simulink model "FullFMS - 2025-11-05 - V0.1"  (R2025b)
settings: Solver=VariableStepAuto  StartTime=0.0  StopTime=inf  RelTol=1e-3
libraries: opcualib x2
settings Model: SimulationMode=accelerator  Creator=guilh  LastModifiedBy=gasie

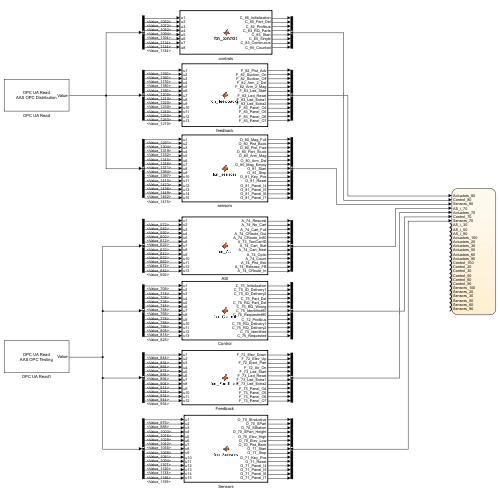
[thumbnail: Simulink's stored preview of the top-level diagram]
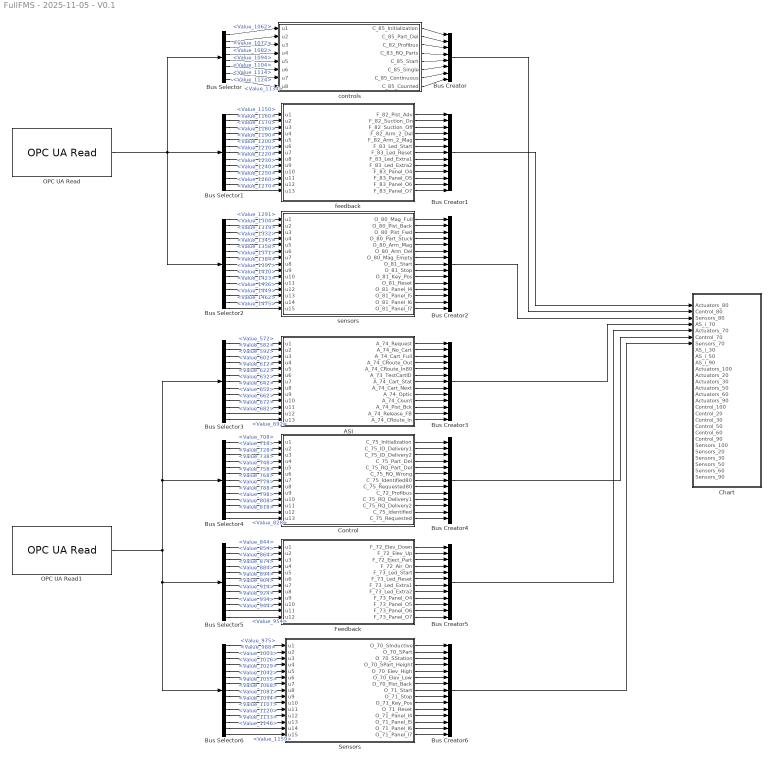
== system FullFMS - 2025-11-05 - V0.1 ==
  ASI : MATLAB Function  TreatAsAtomicUnit=on
  Bus Creator : BusCreator  Inputs=8
  Bus Creator1 : BusCreator  Inputs=13
  Bus Creator2 : BusCreator  Inputs=15
  Bus Creator3 : BusCreator  Inputs=13
  Bus Creator4 : BusCreator  Inputs=13
  Bus Creator5 : BusCreator  Inputs=12
  Bus Creator6 : BusCreator  Inputs=15
  Bus Selector : BusSelector  OutputSignals=Value_1062,Value_1072,Value_1082,Value_1094,Value_1104,Value_1114,Value_1124,Value_1134
  Bus Selector1 : BusSelector  OutputSignals=Value_1150,Value_1160,Value_1170,Value_1180,Value_1190,Value_1200,Value_1210,Value_1220,Value_1230,Value_1240,Value_1250,Value_1260,Value_1270
  Bus Selector2 : BusSelector  OutputSignals=Value_1291,Value_1304,Value_1319,Value_1332,Value_1345,Value_1358,Value_1371,Value_1384,Value_1397,Value_1410,Value_1423,Value_1436,Value_1449,Value_1462,Value_1475
  Bus Selector3 : BusSelector  OutputSignals=Value_572,Value_582,Value_592,Value_602,Value_612,Value_622,Value_632,Value_642,Value_652,Value_662,Value_672,Value_682,Value_692
  Bus Selector4 : BusSelector  OutputSignals=Value_708,Value_718,Value_728,Value_738,Value_748,Value_758,Value_768,Value_778,Value_788,Value_798,Value_808,Value_818,Value_828
  Bus Selector5 : BusSelector  OutputSignals=Value_844,Value_854,Value_864,Value_874,Value_884,Value_894,Value_904,Value_914,Value_924,Value_934,Value_944,Value_954
  Bus Selector6 : BusSelector  OutputSignals=Value_975,Value_988,Value_1003,Value_1016,Value_1029,Value_1042,Value_1055,Value_1068,Value_1081,Value_1094,Value_1107,Value_1120,Value_1133,Value_1146,Value_1159
  Chart : Stateflow chart  TreatAsAtomicUnit=on
      settings: PortSchema="{\"entries\":[{\"content\":{\"sides\":[{\"content\":{\"connectorIds\":[\"In2\",\"In1\",\"In3\",\"In4\",\"In6\",\"In5\",\"In7\",\"In8\",\"In9\",\"In10\",\"In11\",\"In12\",\"In13\",\"In14\",\"In15\",\"In16\",\"In17\",\"In18\",\"In19\",\"In20\",\"In21\",\"In22\",\"In23\",\"In24\",\"In25\",\"In26\",\"In27\",\"In28\"]},\"type\":\"ConnectorPlacement.EquallySpacedRectSide\",\"uuid\":\"e54bf7d4-7c7d-41d9-a8b8-f479ac319a99\"},{\"content\":{\"side\":\"RIGHT\"},\"type\":\"ConnectorPlacement.EquallySpacedRectSide\",\"uuid\":\"d3c20706-71bd-4e26-b40f-0ee7e71b06ee\"},{\"content\":{\"side\":\"TOP\"},\"type\":\"ConnectorPlacement.EquallySpacedRectSide\",\"uuid\":\"ecfb6920-e95b-4ed8-99f9-df5ce878328e\"}]},\"type\":\"ConnectorPlacement.EquallySpacedConnector\",\"uuid\":\"2e714192-4eea-4e1a-8945-7c827feed48f\"}],\"packageUris\":[\"http://schema.mathworks.com/mf0/Connector/R2020b\"],\"version\":\"1.0\"}"
  Control : MATLAB Function  TreatAsAtomicUnit=on
  Feedback : MATLAB Function  TreatAsAtomicUnit=on
  OPC UA Read : opcualib/OPC UA Read  SelectedServer=AAS OPC Distribution  ServerList=AAS OPC Distribution  NodeList={ '1', 'Value', '6', '1062', '1'; '2', 'Value', '6', '1072', '1'; '3', 'Value', '6', '1082', '1'; '4', 'Value', '6', '1094', '1'; '5', 'Value', '6', '1104', '1'; '6', 'Value', '6', '1114', '1'; '7', 'Value', '6', '1124', '1'; '8', 'Value', '6', '1134', '1'; '9', 'Value', '6', '1150', '1'; '10', 'Value', '6', '1160', '1'; '11', 'Value', '6', '1170', '1'; '12', 'Value', '6', '1180', '1'; '13', 'Value', '6', '1190', '1'; '14', 'Value', '6', '1200', '1'; '15', 'Value', '6', '1210', '1'; '16', 'Value', '6', '1220', '1'; '17', 'Value', '6', '1230', '1'; '18', 'Value', '6', '1240', '1'; '19', 'Value', '6', '1250', '1'; '20', 'Value', '6', '1260', '1'; '21', 'Value', '6', '1270', '1'; '22', 'Value', '6', '1291', '1'; '23', 'Value', '6', '1304', '1'; '24', 'Value', '6', '1319', '1'; '25', 'Value', '6', '1332', '1'; '26', 'Value', '6', '1345', '1'; '27', 'Value', '6', '1358', '1'; '28', 'Value', '6', '1371', '1'; '29', 'Value', '6', '1384', '1'; '30', 'Value', '6', '1397', '1'; '31', 'Value', '6', '1410', '1'; '32', 'Value', '6', '1423', '1'; '33', 'Value', '6', '1436', '1'; '34', 'Value', '6', '1449', '1'; '35', 'Value', '6', '1462', '1'; '36', 'Value', '6', '1475', '1' }  ShowQualityPort=off  ShowTimestampPort=off  ShowTimestampPortAs=Seconds since start  SampleTime=-1
  OPC UA Read1 : opcualib/OPC UA Read  SelectedServer=AAS OPC Testing  ServerList=AAS OPC Testing  NodeList={ '1', 'Value', '6', '572', '1'; '2', 'Value', '6', '582', '1'; '3', 'Value', '6', '592', '1'; '4', 'Value', '6', '602', '1'; '5', 'Value', '6', '612', '1'; '6', 'Value', '6', '622', '1'; '7', 'Value', '6', '632', '1'; '8', 'Value', '6', '642', '1'; '9', 'Value', '6', '652', '1'; '10', 'Value', '6', '662', '1'; '11', 'Value', '6', '672', '1'; '12', 'Value', '6', '682', '1'; '13', 'Value', '6', '692', '1'; '14', 'Value', '6', '708', '1'; '15', 'Value', '6', '718', '1'; '16', 'Value', '6', '728', '1'; '17', 'Value', '6', '738', '1'; '18', 'Value', '6', '748', '1'; '19', 'Value', '6', '758', '1'; '20', 'Value', '6', '768', '1'; '21', 'Value', '6', '778', '1'; '22', 'Value', '6', '788', '1'; '23', 'Value', '6', '798', '1'; '24', 'Value', '6', '808', '1'; '25', 'Value', '6', '818', '1'; '26', 'Value', '6', '828', '1'; '27', 'Value', '6', '844', '1'; '28', 'Value', '6', '854', '1'; '29', 'Value', '6', '864', '1'; '30', 'Value', '6', '874', '1'; '31', 'Value', '6', '884', '1'; '32', 'Value', '6', '894', '1'; '33', 'Value', '6', '904', '1'; '34', 'Value', '6', '914', '1'; '35', 'Value', '6', '924', '1'; '36', 'Value', '6', '934', '1'; '37', 'Value', '6', '944', '1'; '38', 'Value', '6', '954', '1'; '39', 'Value', '6', '975', '1'; '40', 'Value', '6', '988', '1'; '41', 'Value', '6', '1003', '1'; '42', 'Value', '6', '1016', '1'; '43', 'Value', '6', '1029', '1'; '44', 'Value', '6', '1042', '1'; '45', 'Value', '6', '1055', '1'; '46', 'Value', '6', '1068', '1'; '47', 'Value', '6', '1081', '1'; '48', 'Value', '6', '1094', '1'; '49', 'Value', '6', '1107', '1'; '50', 'Value', '6', '1120', '1'; '51', 'Value', '6', '1133', '1'; '52', 'Value', '6', '1146', '1'; '53', 'Value', '6', '1159', '1' }  ShowQualityPort=off  ShowTimestampPort=off  ShowTimestampPortAs=Seconds since start  SampleTime=-1
  Sensors : MATLAB Function  TreatAsAtomicUnit=on
  controls : MATLAB Function  TreatAsAtomicUnit=on
  feedback : MATLAB Function  TreatAsAtomicUnit=on
  sensors : MATLAB Function  TreatAsAtomicUnit=on
  wires:
  OPC UA Read/1 -> Bus Selector2/1, Bus Selector/1, Bus Selector1/1
  Bus Selector/1 -> controls/1(u1)  "<Value_1062>"
  Bus Selector/2 -> controls/2(u2)  "<Value_1072>"
  Bus Selector/3 -> controls/3(u3)  "<Value_1082>"
  Bus Selector/4 -> controls/4(u4)  "<Value_1094>"
  Bus Selector/5 -> controls/5(u5)  "<Value_1104>"
  Bus Selector/6 -> controls/6(u6)  "<Value_1114>"
  Bus Selector/7 -> controls/7(u7)  "<Value_1124>"
  Bus Selector/8 -> controls/8(u8)  "<Value_1134>"
  Bus Selector1/11 -> feedback/11(u11)  "<Value_1250>"
  Bus Selector1/12 -> feedback/12(u12)  "<Value_1260>"
  Bus Selector1/13 -> feedback/13(u13)  "<Value_1270>"
  Bus Selector1/1 -> feedback/1(u1)  "<Value_1150>"
  Bus Selector1/2 -> feedback/2(u2)  "<Value_1160>"
  Bus Selector1/3 -> feedback/3(u3)  "<Value_1170>"
  Bus Selector1/4 -> feedback/4(u4)  "<Value_1180>"
  Bus Selector1/5 -> feedback/5(u5)  "<Value_1190>"
  Bus Selector1/6 -> feedback/6(u6)  "<Value_1200>"
  Bus Selector1/7 -> feedback/7(u7)  "<Value_1210>"
  Bus Selector1/8 -> feedback/8(u8)  "<Value_1220>"
  Bus Selector1/9 -> feedback/9(u9)  "<Value_1230>"
  Bus Selector1/10 -> feedback/10(u10)  "<Value_1240>"
  Bus Selector2/1 -> sensors/1(u1)  "<Value_1291>"
  Bus Selector2/2 -> sensors/2(u2)  "<Value_1304>"
  Bus Selector2/3 -> sensors/3(u3)  "<Value_1319>"
  Bus Selector2/4 -> sensors/4(u4)  "<Value_1332>"
  Bus Selector2/5 -> sensors/5(u5)  "<Value_1345>"
  Bus Selector2/6 -> sensors/6(u6)  "<Value_1358>"
  Bus Selector2/7 -> sensors/7(u7)  "<Value_1371>"
  Bus Selector2/8 -> sensors/8(u8)  "<Value_1384>"
  Bus Selector2/9 -> sensors/9(u9)  "<Value_1397>"
  Bus Selector2/10 -> sensors/10(u10)  "<Value_1410>"
  Bus Selector2/11 -> sensors/11(u11)  "<Value_1423>"
  Bus Selector2/12 -> sensors/12(u12)  "<Value_1436>"
  Bus Selector2/13 -> sensors/13(u13)  "<Value_1449>"
  Bus Selector2/14 -> sensors/14(u14)  "<Value_1462>"
  Bus Selector2/15 -> sensors/15(u15)  "<Value_1475>"
  OPC UA Read1/1 -> Bus Selector6/1, Bus Selector5/1, Bus Selector3/1, Bus Selector4/1
  Bus Selector3/1 -> ASI/1(u1)  "<Value_572>"
  Bus Selector3/2 -> ASI/2(u2)  "<Value_582>"
  Bus Selector3/3 -> ASI/3(u3)  "<Value_592>"
  Bus Selector3/4 -> ASI/4(u4)  "<Value_602>"
  Bus Selector3/5 -> ASI/5(u5)  "<Value_612>"
  Bus Selector3/6 -> ASI/6(u6)  "<Value_622>"
  Bus Selector3/7 -> ASI/7(u7)  "<Value_632>"
  Bus Selector3/8 -> ASI/8(u8)  "<Value_642>"
  Bus Selector3/9 -> ASI/9(u9)  "<Value_652>"
  Bus Selector3/10 -> ASI/10(u10)  "<Value_662>"
  Bus Selector3/11 -> ASI/11(u11)  "<Value_672>"
  Bus Selector3/12 -> ASI/12(u12)  "<Value_682>"
  Bus Selector3/13 -> ASI/13(u13)  "<Value_692>"
  Bus Selector4/1 -> Control/1(u1)  "<Value_708>"
  Bus Selector4/2 -> Control/2(u2)  "<Value_718>"
  Bus Selector4/3 -> Control/3(u3)  "<Value_728>"
  Bus Selector4/4 -> Control/4(u4)  "<Value_738>"
  Bus Selector4/5 -> Control/5(u5)  "<Value_748>"
  Bus Selector4/6 -> Control/6(u6)  "<Value_758>"
  Bus Selector4/7 -> Control/7(u7)  "<Value_768>"
  Bus Selector4/8 -> Control/8(u8)  "<Value_778>"
  Bus Selector4/9 -> Control/9(u9)  "<Value_788>"
  Bus Selector4/10 -> Control/10(u10)  "<Value_798>"
  Bus Selector4/11 -> Control/11(u11)  "<Value_808>"
  Bus Selector4/12 -> Control/12(u12)  "<Value_818>"
  Bus Selector4/13 -> Control/13(u13)  "<Value_828>"
  Bus Selector5/1 -> Feedback/1(u1)  "<Value_844>"
  Bus Selector5/2 -> Feedback/2(u2)  "<Value_854>"
  Bus Selector5/3 -> Feedback/3(u3)  "<Value_864>"
  Bus Selector5/4 -> Feedback/4(u4)  "<Value_874>"
  Bus Selector5/5 -> Feedback/5(u5)  "<Value_884>"
  Bus Selector5/6 -> Feedback/6(u6)  "<Value_894>"
  Bus Selector5/7 -> Feedback/7(u7)  "<Value_904>"
  Bus Selector5/8 -> Feedback/8(u8)  "<Value_914>"
  Bus Selector5/9 -> Feedback/9(u9)  "<Value_924>"
  Bus Selector5/10 -> Feedback/10(u10)  "<Value_934>"
  Bus Selector5/11 -> Feedback/11(u11)  "<Value_944>"
  Bus Selector5/12 -> Feedback/12(u12)  "<Value_954>"
  Bus Selector6/1 -> Sensors/1(u1)  "<Value_975>"
  Bus Selector6/2 -> Sensors/2(u2)  "<Value_988>"
  Bus Selector6/3 -> Sensors/3(u3)  "<Value_1003>"
  Bus Selector6/4 -> Sensors/4(u4)  "<Value_1016>"
  Bus Selector6/5 -> Sensors/5(u5)  "<Value_1029>"
  Bus Selector6/6 -> Sensors/6(u6)  "<Value_1042>"
  Bus Selector6/7 -> Sensors/7(u7)  "<Value_1055>"
  Bus Selector6/8 -> Sensors/8(u8)  "<Value_1068>"
  Bus Selector6/9 -> Sensors/9(u9)  "<Value_1081>"
  Bus Selector6/10 -> Sensors/10(u10)  "<Value_1094>"
  Bus Selector6/11 -> Sensors/11(u11)  "<Value_1107>"
  Bus Selector6/12 -> Sensors/12(u12)  "<Value_1120>"
  Bus Selector6/13 -> Sensors/13(u13)  "<Value_1133>"
  Bus Selector6/14 -> Sensors/14(u14)  "<Value_1146>"
  Bus Selector6/15 -> Sensors/15(u15)  "<Value_1159>"
  controls/1(C_85_Initialization) -> Bus Creator/1
  controls/2(C_85_Part_Del) -> Bus Creator/2
  controls/3(C_82_Profibus) -> Bus Creator/3
  controls/4(C_83_RQ_Parts) -> Bus Creator/4
  controls/5(C_85_Start) -> Bus Creator/5
  controls/6(C_85_Single) -> Bus Creator/6
  controls/7(C_85_Continuous) -> Bus Creator/7
  controls/8(C_85_Counted) -> Bus Creator/8
  feedback/1(F_82_Pist_Adv) -> Bus Creator1/1
  feedback/2(F_82_Suction_On) -> Bus Creator1/2
  feedback/3(F_82_Suction_Off) -> Bus Creator1/3
  feedback/4(F_82_Arm_2_Del) -> Bus Creator1/4
  feedback/5(F_82_Arm_2_Mag) -> Bus Creator1/5
  feedback/6(F_83_Led_Start) -> Bus Creator1/6
  feedback/7(F_83_Led_Reset) -> Bus Creator1/7
  feedback/8(F_83_Led_Extra1) -> Bus Creator1/8
  feedback/9(F_83_Led_Extra2) -> Bus Creator1/9
  feedback/10(F_83_Panel_O4) -> Bus Creator1/10
  feedback/11(F_83_Panel_O5) -> Bus Creator1/11
  feedback/12(F_83_Panel_O6) -> Bus Creator1/12
  feedback/13(F_83_Panel_O7) -> Bus Creator1/13
  sensors/1(O_80_Mag_Full) -> Bus Creator2/1
  sensors/2(O_80_Pist_Back) -> Bus Creator2/2
  sensors/3(O_80_Pist_Fwd) -> Bus Creator2/3
  sensors/4(O_80_Part_Stuck) -> Bus Creator2/4
  sensors/5(O_80_Arm_Mag) -> Bus Creator2/5
  sensors/6(O_80_Arm_Del) -> Bus Creator2/6
  sensors/7(O_80_Mag_Empty) -> Bus Creator2/7
  sensors/8(O_81_Start) -> Bus Creator2/8
  sensors/9(O_81_Stop) -> Bus Creator2/9
  sensors/10(O_81_Key_Pos) -> Bus Creator2/10
  sensors/11(O_81_Reset) -> Bus Creator2/11
  sensors/12(O_81_Panel_I4) -> Bus Creator2/12
  sensors/13(O_81_Panel_I5) -> Bus Creator2/13
  sensors/14(O_81_Panel_I6) -> Bus Creator2/14
  sensors/15(O_81_Panel_I7) -> Bus Creator2/15
  ASI/1(A_74_Request) -> Bus Creator3/1
  ASI/2(A_74_No_Cart) -> Bus Creator3/2
  ASI/3(A_74_Cart_Full) -> Bus Creator3/3
  ASI/4(A_74_CRoute_Out) -> Bus Creator3/4
  ASI/5(A_74_CRoute_In80) -> Bus Creator3/5
  ASI/6(A_73_TestCartID) -> Bus Creator3/6
  ASI/7(A_74_Cart_Stat) -> Bus Creator3/7
  ASI/8(A_74_Cart_Next) -> Bus Creator3/8
  ASI/9(A_74_Optic) -> Bus Creator3/9
  ASI/10(A_74_Count) -> Bus Creator3/10
  ASI/11(A_74_Pist_Bck) -> Bus Creator3/11
  ASI/12(A_74_Release_FB) -> Bus Creator3/12
  ASI/13(A_74_CRoute_In) -> Bus Creator3/13
  Control/1(C_75_Initialization) -> Bus Creator4/1
  Control/2(C_75_ID_Delivery1) -> Bus Creator4/2
  Control/3(C_75_ID_Delivery2) -> Bus Creator4/3
  Control/4(C_75_Part_Del) -> Bus Creator4/4
  Control/5(C_75_RQ_Part_Del) -> Bus Creator4/5
  Control/6(C_75_RQ_Wrong) -> Bus Creator4/6
  Control/7(C_75_Identified80) -> Bus Creator4/7
  Control/8(C_75_Requested80) -> Bus Creator4/8
  Control/9(C_72_Profibus) -> Bus Creator4/9
  Control/10(C_75_RQ_Delivery1) -> Bus Creator4/10
  Control/11(C_75_RQ_Delivery2) -> Bus Creator4/11
  Control/12(C_75_Identified) -> Bus Creator4/12
  Control/13(C_75_Requested) -> Bus Creator4/13
  Feedback/1(F_72_Elev_Down) -> Bus Creator5/1
  Feedback/2(F_72_Elev_Up) -> Bus Creator5/2
  Feedback/3(F_72_Eject_Part) -> Bus Creator5/3
  Feedback/4(F_72_Air_On) -> Bus Creator5/4
  Feedback/5(F_73_Led_Start) -> Bus Creator5/5
  Feedback/6(F_73_Led_Reset) -> Bus Creator5/6
  Feedback/7(F_73_Led_Extra1) -> Bus Creator5/7
  Feedback/8(F_73_Led_Extra2) -> Bus Creator5/8
  Feedback/9(F_73_Panel_O4) -> Bus Creator5/9
  Feedback/10(F_73_Panel_O5) -> Bus Creator5/10
  Feedback/11(F_73_Panel_O6) -> Bus Creator5/11
  Feedback/12(F_73_Panel_O7) -> Bus Creator5/12
  Sensors/1(O_70_SInductive) -> Bus Creator6/1
  Sensors/2(O_70_SPart) -> Bus Creator6/2
  Sensors/3(O_70_SStation) -> Bus Creator6/3
  Sensors/4(O_70_SPart_Height) -> Bus Creator6/4
  Sensors/5(O_70_Elev_High) -> Bus Creator6/5
  Sensors/6(O_70_Elev_Low) -> Bus Creator6/6
  Sensors/7(O_70_Pist_Back) -> Bus Creator6/7
  Sensors/8(O_71_Start) -> Bus Creator6/8
  Sensors/9(O_71_Stop) -> Bus Creator6/9
  Sensors/10(O_71_Key_Pos) -> Bus Creator6/10
  Sensors/11(O_71_Reset) -> Bus Creator6/11
  Sensors/12(O_71_Panel_I4) -> Bus Creator6/12
  Sensors/13(O_71_Panel_I5) -> Bus Creator6/13
  Sensors/14(O_71_Panel_I6) -> Bus Creator6/14
  Sensors/15(O_71_Panel_I7) -> Bus Creator6/15
  Bus Creator/1 -> Chart/1(Control_80)
  Bus Creator1/1 -> Chart/2(Actuators_80)
  Bus Creator2/1 -> Chart/3(Sensors_80)
  Bus Creator6/1 -> Chart/7(Sensors_70)
  Bus Creator5/1 -> Chart/6(Actuators_70)
  Bus Creator4/1 -> Chart/5(Control_70)
  Bus Creator3/1 -> Chart/4(AS_i_70)

== matlab function FullFMS - 2025-11-05 - V0.1/feedback ==
  data: u1 input; F_82_Pist_Adv output; u2 input; u3 input; u4 input; u5 input; u6 input; u7 input; u8 input; u9 input; u10 input; u11 input; u12 input; u13 input; F_82_Suction_On output; F_82_Suction_Off output; F_82_Arm_2_Del output; F_82_Arm_2_Mag output; F_83_Led_Start output; F_83_Led_Reset output; F_83_Led_Extra1 output; F_83_Led_Extra2 output; F_83_Panel_O4 output; F_83_Panel_O5 output; F_83_Panel_O6 output; F_83_Panel_O7 output
function [F_82_Pist_Adv,F_82_Suction_On,F_82_Suction_Off,F_82_Arm_2_Del, ...
    F_82_Arm_2_Mag,F_83_Led_Start,F_83_Led_Reset,F_83_Led_Extra1,...
    F_83_Led_Extra2,F_83_Panel_O4,F_83_Panel_O5,F_83_Panel_O6,...
    F_83_Panel_O7] = fcn_feedbacks(u1,u2,u3,u4,u5,u6,u7,u8,u9,...
    u10,u11,u12,u13)

F_82_Pist_Adv = u1;
F_82_Suction_On = u2;
F_82_Suction_Off = u3;
F_82_Arm_2_Del = u4;
F_82_Arm_2_Mag = u5;
F_83_Led_Start = u6;
F_83_Led_Reset = u7;
F_83_Led_Extra1 = u8;
F_83_Led_Extra2 = u9;
F_83_Panel_O4 = u10;
F_83_Panel_O5 = u11;
F_83_Panel_O6 = u12;
F_83_Panel_O7 = u13;

== matlab function FullFMS - 2025-11-05 - V0.1/controls ==
  data: C_85_Initialization output; C_85_Part_Del output; u1 input; u2 input; u3 input; u4 input; u5 input; u6 input; u7 input; C_82_Profibus output; C_83_RQ_Parts output; C_85_Start output; C_85_Single output; C_85_Continuous output; C_85_Counted output; u8 input
function [C_85_Initialization, C_85_Part_Del,...
    C_82_Profibus, C_83_RQ_Parts, ...
    C_85_Start,C_85_Single, C_85_Continuous, ...
    C_85_Counted] = fcn_controls(u1,u2,u3,u4,u5,u6,u7,u8)

C_85_Initialization = u1;
C_85_Part_Del = u2;
C_82_Profibus = u3;
C_83_RQ_Parts = u4;
C_85_Start = u5;
C_85_Single = u6; 
C_85_Continuous = u7;
C_85_Counted = u8;

== matlab function FullFMS - 2025-11-05 - V0.1/ASI ==
  data: u1 input; A_74_Request output; u2 input; u3 input; u4 input; u5 input; u6 input; u7 input; u8 input; u9 input; A_74_No_Cart output; A_74_Cart_Full output; A_74_CRoute_Out output; A_74_CRoute_In80 output; A_73_TestCartID output; A_74_Cart_Stat output; A_74_Cart_Next output; A_74_Optic output; A_74_Count output; A_74_Pist_Bck output; A_74_Release_FB output; A_74_CRoute_In output; u10 input; u11 input; u12 input; u13 input
function [A_74_Request, A_74_No_Cart, A_74_Cart_Full, A_74_CRoute_Out,...
    A_74_CRoute_In80, A_73_TestCartID, A_74_Cart_Stat, ...
          A_74_Cart_Next, A_74_Optic, A_74_Count, A_74_Pist_Bck, ...
          A_74_Release_FB,...
          A_74_CRoute_In] = fcn_Asi(u1, u2, u3, u4, u5, u6, u7, u8, u9,...
          u10, u11, u12, u13)

A_74_Request = u1;
A_74_No_Cart = u2;
A_74_Cart_Full = u3;
A_74_CRoute_Out = u4;
A_74_CRoute_In80 = u5;
A_73_TestCartID = u6;
A_74_Cart_Stat = u7;
A_74_Cart_Next = u8;
A_74_Optic = u9;
A_74_Count = u10;
A_74_Pist_Bck = u11;
A_74_Release_FB = u12;
A_74_CRoute_In = u13;

== matlab function FullFMS - 2025-11-05 - V0.1/sensors ==
  data: u1 input; u2 input; u3 input; u4 input; u5 input; u6 input; u7 input; u8 input; u9 input; u10 input; u11 input; u12 input; u13 input; u14 input; u15 input; O_80_Mag_Full output; O_80_Pist_Back output; O_80_Pist_Fwd output; O_80_Part_Stuck output; O_80_Arm_Mag output; O_80_Arm_Del output; O_80_Mag_Empty output; O_81_Start output; O_81_Stop output; O_81_Key_Pos output; O_81_Reset output; O_81_Panel_I4 output; O_81_Panel_I5 output; O_81_Panel_I6 output; O_81_Panel_I7 output
function [O_80_Mag_Full,O_80_Pist_Back,O_80_Pist_Fwd,O_80_Part_Stuck,...
    O_80_Arm_Mag,O_80_Arm_Del,O_80_Mag_Empty,O_81_Start,O_81_Stop,...
    O_81_Key_Pos,O_81_Reset,O_81_Panel_I4,O_81_Panel_I5,O_81_Panel_I6,...
    O_81_Panel_I7] = fcn_sensors(u1,u2,u3,u4,u5,u6,u7,u8,u9,...
    u10,u11,u12,u13,u14,u15)

O_80_Mag_Full = u1;
O_80_Pist_Back = u2;
O_80_Pist_Fwd = u3;
O_80_Part_Stuck = u4;
O_80_Arm_Mag = u5;
O_80_Arm_Del = u6;
O_80_Mag_Empty = u7;
O_81_Start = u8;
O_81_Stop = u9;
O_81_Key_Pos = u10;
O_81_Reset = u11;
O_81_Panel_I4 = u12;
O_81_Panel_I5 = u13;
O_81_Panel_I6 = u14;
O_81_Panel_I7 = u15;

== matlab function FullFMS - 2025-11-05 - V0.1/Control ==
  data: C_75_Initialization output; C_75_ID_Delivery1 output; C_75_ID_Delivery2 output; C_75_Part_Del output; C_75_RQ_Part_Del output; C_75_RQ_Wrong output; C_75_Identified80 output; C_75_Requested80 output; u1 input; C_72_Profibus output; u2 input; u3 input; u4 input; u5 input; u6 input; u7 input; u8 input; u9 input; u10 input; u11 input; u12 input; u13 input; C_75_RQ_Delivery1 output; C_75_RQ_Delivery2 output; C_75_Identified output; C_75_Requested output
function [C_75_Initialization, C_75_ID_Delivery1, C_75_ID_Delivery2, ...
          C_75_Part_Del, C_75_RQ_Part_Del, C_75_RQ_Wrong, C_75_Identified80, ...
          C_75_Requested80, C_72_Profibus, C_75_RQ_Delivery1, C_75_RQ_Delivery2, C_75_Identified, ...
          C_75_Requested] = fcn_Control(u1, u2, u3, u4, u5, u6, u7, u8, u9, u10, u11, u12, u13)

C_75_Initialization = u1;
C_75_ID_Delivery1 = u2;
C_75_ID_Delivery2 = u3;
C_75_Part_Del = u4;
C_75_RQ_Part_Del = u5;
C_75_RQ_Wrong = u6;
C_75_Identified80 = u7;
C_75_Requested80 = u8;
C_72_Profibus = u9;
C_75_RQ_Delivery1 = u10;
C_75_RQ_Delivery2 = u11;
C_75_Identified = u12;
C_75_Requested = u13;

== matlab function FullFMS - 2025-11-05 - V0.1/Feedback ==
  data: u1 input; F_72_Elev_Down output; u2 input; u3 input; u4 input; u5 input; u6 input; u7 input; u8 input; u9 input; u10 input; u11 input; u12 input; F_72_Elev_Up output; F_72_Eject_Part output; F_72_Air_On output; F_73_Led_Start output; F_73_Led_Reset output; F_73_Led_Extra1 output; F_73_Led_Extra2 output; F_73_Panel_O4 output; F_73_Panel_O5 output; F_73_Panel_O6 output; F_73_Panel_O7 output
function [F_72_Elev_Down, F_72_Elev_Up, F_72_Eject_Part, F_72_Air_On, ...
          F_73_Led_Start, F_73_Led_Reset, F_73_Led_Extra1, F_73_Led_Extra2, ...
          F_73_Panel_O4, F_73_Panel_O5, F_73_Panel_O6, F_73_Panel_O7] = ...
          fcn_Feedback(u1, u2, u3, u4, u5, u6, u7, u8, u9, u10, u11, u12)

F_72_Elev_Down = u1;
F_72_Elev_Up = u2;
F_72_Eject_Part = u3;
F_72_Air_On = u4;
F_73_Led_Start = u5;
F_73_Led_Reset = u6;
F_73_Led_Extra1 = u7;
F_73_Led_Extra2 = u8;
F_73_Panel_O4 = u9;
F_73_Panel_O5 = u10;
F_73_Panel_O6 = u11;
F_73_Panel_O7 = u12;

== matlab function FullFMS - 2025-11-05 - V0.1/Sensors ==
  data: u1 input; O_70_SInductive output; u2 input; u3 input; u4 input; u5 input; u6 input; u7 input; u8 input; u9 input; u10 input; u11 input; u12 input; u13 input; u14 input; u15 input; O_70_SPart output; O_70_SStation output; O_70_SPart_Height output; O_70_Elev_High output; O_70_Elev_Low output; O_70_Pist_Back output; O_71_Start output; O_71_Stop output; O_71_Key_Pos output; O_71_Reset output; O_71_Panel_I4 output; O_71_Panel_I5 output; O_71_Panel_I6 output; O_71_Panel_I7 output
function [O_70_SInductive, O_70_SPart, O_70_SStation, O_70_SPart_Height, ...
          O_70_Elev_High, O_70_Elev_Low, O_70_Pist_Back, O_71_Start, ...
          O_71_Stop, O_71_Key_Pos, O_71_Reset, O_71_Panel_I4, O_71_Panel_I5, ...
          O_71_Panel_I6, O_71_Panel_I7] = ...
          fcn_Sensors(u1, u2, u3, u4, u5, u6, u7, u8, u9, u10, ...
          u11, u12, u13, u14, u15)

O_70_SInductive = u1;
O_70_SPart = u2;
O_70_SStation = u3;
O_70_SPart_Height = u4;
O_70_Elev_High = u5;
O_70_Elev_Low = u6;
O_70_Pist_Back = u7;
O_71_Start = u8;
O_71_Stop = u9;
O_71_Key_Pos = u10;
O_71_Reset = u11;
O_71_Panel_I4 = u12;
O_71_Panel_I5 = u13;
O_71_Panel_I6 = u14;
O_71_Panel_I7 = u15;

== stateflow chart FullFMS - 2025-11-05 - V0.1/Chart ==
  state VarDeclaration_60
    entry:
    %Control_60
    C_65_Initialization = Control_60(1);
    C_65_ID_1           = Control_60(2);
    C_65_ID_2           = Control_60(3);
    C_62_Profibus       = Control_60(4);
    C_65_RBS_Output     = Control_60(5);
    C_65_RSB_Output     = Control_60(6);
    C_65_BRS_Output     = Control_60(7);
    C_65_BSR_Output     = Control_60(8);
    C_65_SRB_Output     = Control_60(9);
    C_65_SBR_Output     = Control_60(10);
    %Actuators_60
    F_62_Conveyor   = Actuators_60(1);
    F_62_P1         = Actuators_60(2);
    F_62_P2         = Actuators_60(3);
    F_62_Identify   = Actuators_60(4);
    F_63_Led_Start  = Actuators_60(5);
    F_63_Led_Reset  = Actuators_60(6);
    F_63_Led_Extra1 = Actuators_60(7);
    F_63_Led_Extra2 = Actuators_60(8);
    F_63_Panel_O4   = Actuators_60(9);
    F_63_Panel_O5   = Actuators_60(10);
    F_63_Panel_O6   = Actuators_60(11);
    F_63_Panel_O7   = Actuators_60(12);
    %Sensors_60
    O_60_SPart      = Sensors_60(1);
    O_60_Slnd       = Sensors_60(2);
    O_60_SPhoto     = Sensors_60(3);
    O_60_Part_Pass  = Sensors_60(4);
    O_60_SL1_Bck    = Sensors_60(5);
    O_60_SL1_Fwd    = Sensors_60(6);
    O_60_SL2_Bck    = Sensors_60(7);
    O_60_SL2_Fwd    = Sensors_60(8);
    O_61_Start      = Sensors_60(9);
    O_61_Stop       = Sensors_60(10);
    O_61_Key_Pos    = Sensors_60(11);
    O_61_Reset      = Sensors_60(12);
    O_61_Panel_I4   = Sensors_60(13);
    O_61_Panel_I5   = Sensors_60(14);
    O_61_Panel_I6   = Sensors_60(15);
    O_61_Panel_I7   = Sensors_60(16);
  state VarDeclaration_70
    entry:
    %AS_i_70
    A_74_Request = AS_i_70(1);
    A_74_No_Cart = AS_i_70(2);
    A_74_Cart_Full = AS_i_70(3);
    A_74_CRoute_Out = AS_i_70(4);
    A_74_CRoute_In80 = AS_i_70(5);
    A_73_TestCartID = AS_i_70(6);
    A_74_Cart_Stat = AS_i_70(7);
    A_74_Cart_Next = AS_i_70(8);
    A_74_Optic = AS_i_70(9);
    A_74_Count = AS_i_70(10);
    A_74_Pist_Bck = AS_i_70(11);
    A_74_Release_FB = AS_i_70(12);
    A_74_CRoute_In = AS_i_70(13);
    %Control_70
    C_75_Initialization = Control_70(1);
    C_75_ID_Delivery1 = Control_70(2);
    C_75_ID_Delivery2 = Control_70(3);
    C_75_Part_Del = Control_70(4);
    C_75_RQ_Part_Del = Control_70(5);
    C_75_RQ_Wrong = Control_70(6);
    C_75_Identified80 = Control_70(7);
    C_75_Requested80 = Control_70(8);
    C_72_Profibus = Control_70(9);
    C_75_RQ_Delivery1 = Control_70(10);
    C_75_RQ_Delivery2 = Control_70(11);
    C_75_Identified = Control_70(12);
    C_75_Requested = Control_70(13);
    %Actuators_70
    F_72_Elev_Down = Actuators_70(1);
    F_72_Elev_Up = Actuators_70(2);
    F_72_Eject_Part = Actuators_70(3);
    F_72_Air_On = Actuators_70(4);
    F_73_Led_Start = Actuators_70(5);
    F_73_Led_Reset = Actuators_70(6);
    F_73_Led_Extra1 = Actuators_70(7);
    F_73_Led_Extra2 = Actuators_70(8);
    F_73_Panel_O4 = Actuators_70(9);
    F_73_Panel_O5 = Actuators_70(10);
    F_73_Panel_O6 = Actuators_70(11);
    F_73_Panel_O7 = Actuators_70(12);
    %Sensors_70
    O_70_SInductive = Sensors_70(1);
    O_70_SPart = Sensors_70(2);
    O_70_SStation = Sensors_70(3);
    O_70_SPart_Height = Sensors_70(4);
    O_70_Elev_High = Sensors_70(5);
    O_70_Elev_Low = Sensors_70(6);
    O_70_Pist_Back = Sensors_70(7);
    O_71_Start = Sensors_70(8);
    O_71_Stop = Sensors_70(9);
    O_71_Key_Pos = Sensors_70(10);
    O_71_Reset = Sensors_70(11);
    O_71_Panel_I4 = Sensors_70(12);
    O_71_Panel_I5 = Sensors_70(13);
    O_71_Panel_I6 = Sensors_70(14);
    O_71_Panel_I7 = Sensors_70(15);
  state VarDeclaration_80
    entry:
    %Control_80
    C_85_Initialization = Control_80(1);
    C_85_Part_Del = Control_80(2);
    C_82_Profibus = Control_80(3);
    C_83_RQ_Parts = Control_80(4);
    C_85_Start = Control_80(5);
    C_85_Single = Control_80(6);
    C_85_Continuous = Control_80(7);
    C_85_Counted = Control_80(8);
    %Actuators_80
    F_82_Pist_Adv = Actuators_80(1);
    F_82_Suction_On = Actuators_80(2);
    F_82_Suction_Off = Actuators_80(3);
    F_82_Arm_2_Del = Actuators_80(4);
    F_82_Arm_2_Mag = Actuators_80(5);
    F_83_Led_Start = Actuators_80(6);
    F_83_Led_Reset = Actuators_80(7);
    F_83_Led_Extra1 = Actuators_80(8);
    F_83_Led_Extra2 = Actuators_80(9);
    F_83_Panel_O4 = Actuators_80(10);
    F_83_Panel_O5 = Actuators_80(11);
    F_83_Panel_O6 = Actuators_80(12);
    F_83_Panel_O7 = Actuators_80(13);
    %Sensors_80
    O_80_Mag_Full = Sensors_80(1);
    O_80_Pist_Back = Sensors_80(2);
    O_80_Pist_Fwd = Sensors_80(3);
    O_80_Part_Stuck = Sensors_80(4);
    O_80_Arm_Mag = Sensors_80(5);
    O_80_Arm_Del = Sensors_80(6);
    O_80_Mag_Empty = Sensors_80(7);
    O_81_Start = Sensors_80(8);
    O_81_Stop = Sensors_80(9);
    O_81_Key_Pos = Sensors_80(10);
    O_81_Reset = Sensors_80(11);
    O_81_Panel_I4 = Sensors_80(12);
    O_81_Panel_I5 = Sensors_80(13);
    O_81_Panel_I6 = Sensors_80(14);
    O_81_Panel_I7 = Sensors_80(15);
  state VarDeclaration_90
    entry:
    %AS_i_90
    A_94_Request    = AS_i_90(1);
    A_94_No_Cart    = AS_i_90(2);
    A_94_Cart_Full  = AS_i_90(3);
    A_94_CRoute_Out = AS_i_90(4);
    A_93_ProcCartID = AS_i_90(5);
    A_94_Cart_Stat  = AS_i_90(6);
    A_94_Cart_Next  = AS_i_90(7);
    A_94_Optic      = AS_i_90(8);
    A_94_Count      = AS_i_90(9);
    A_94_Pist_Bck   = AS_i_90(10);
    A_94_Release_FB = AS_i_90(11);
    A_94_CRoute_In  = AS_i_90(12);
    %Control_90
    C_95_Initialization = Control_90(1);
    C_95_PD_Proc        = Control_90(2);
    C_95_PD_Cart        = Control_90(3);
    C_92_Profibus       = Control_90(4);
    C_95_Start          = Control_90(5);
    C_95_Cart2Del       = Control_90(6);
    C_95_Del2Cart       = Control_90(7);
    %Actuators_90
    F_92_Claw_2_Cart = Actuators_90(1);
    F_92_Claw_2_Del  = Actuators_90(2);
    F_92_Claw_Down   = Actuators_90(3);
    F_92_Close_Claw  = Actuators_90(4);
    F_93_Led_Start   = Actuators_90(5);
    F_93_Led_Reset   = Actuators_90(6);
    F_93_Led_Extra1  = Actuators_90(7);
    F_93_Led_Extra2  = Actuators_90(8);
    F_93_Panel_O4    = Actuators_90(9);
    F_93_Panel_O5    = Actuators_90(10);
    F_93_Panel_O6    = Actuators_90(11);
    F_93_Panel_O7    = Actuators_90(12);
    %Sensors_90
    O_90_Part_Reserve = Sensors_90(1);
    O_90_Claw_Del     = Sensors_90(2);
    O_90_Claw_Cart    = Sensors_90(3);
    O_90_Claw_Reserve = Sensors_90(4);
    O_90_Claw_Low     = Sensors_90(5);
    O_90_Claw_High    = Sensors_90(6);
    O_90_Part_in_Claw = Sensors_90(7);
    O_91_Start        = Sensors_90(8);
    O_91_Stop         = Sensors_90(9);
    O_91_Key_Pos      = Sensors_90(10);
    O_91_Reset        = Sensors_90(11);
    O_91_Panel_I4     = Sensors_90(12);
    O_91_Panel_I5     = Sensors_90(13);
    O_91_Panel_I6     = Sensors_90(14);
    O_91_Panel_I7     = Sensors_90(15);
  state VarDeclaration_100
    entry:
    %Control_100
    C_105_Initialization = Control_100(1);
    C_105_Part_ready     = Control_100(2);
    C_105_Test_Ok        = Control_100(3);
    C_105_Test_Fail      = Control_100(4);
    C_102_Profibus       = Control_100(5);
    C_103_RQ_Turns       = Control_100(6);
    C_105_Start          = Control_100(7);
    C_105_Test           = Control_100(8);
    C_105_TestDrill      = Control_100(9);
    C_105_Rotation       = Control_100(10);
    %Actuators_100
    F_102_Drill_On   = Actuators_100(1);
    F_102_RT_On      = Actuators_100(2);
    F_102_Drill_Down = Actuators_100(3);
    F_102_Drill_Up   = Actuators_100(4);
    F_102_Drill_Pin  = Actuators_100(5);
    F_102_Test_Pin   = Actuators_100(6);
    F_103_Led_Start  = Actuators_100(7);
    F_103_Led_Reset  = Actuators_100(8);
    F_103_Led_Extra1 = Actuators_100(9);
    F_103_Led_Extra2 = Actuators_100(10);
    F_103_Panel_O4   = Actuators_100(11);
    F_103_Panel_O5   = Actuators_100(12);
    F_103_Panel_O6   = Actuators_100(13);
    F_103_Panel_O7   = Actuators_100(14);
    %Sensors_100
    O_100_PInit_Pos   = Sensors_100(1);
    O_100_PDrill_Pos  = Sensors_100(2);
    O_100_PTest_Pos   = Sensors_100(3);
    O_100_SDrill_High = Sensors_100(4);
    O_100_SDrill_Low  = Sensors_100(5);
    O_100_RT_Sensor   = Sensors_100(6);
    O_100_PTest_Ok    = Sensors_100(7);
    O_101_Start       = Sensors_100(8);
    O_101_Stop        = Sensors_100(9);
    O_101_Key_Pos     = Sensors_100(10);
    O_101_Reset       = Sensors_100(11);
    O_101_Panel_I4    = Sensors_100(12);
    O_101_Panel_I5    = Sensors_100(13);
    O_101_Panel_I6    = Sensors_100(14);
    O_101_Panel_I7    = Sensors_100(15);
  state VarDeclaration_50
    entry:
    %AS_i_50
    A_54_Request    = AS_i_50(1);
    A_54_No_Cart    = AS_i_50(2);
    A_54_Cart_Full  = AS_i_50(3);
    A_54_CRoute_Out = AS_i_50(4);
    A_53_SortCartID = AS_i_50(5);
    A_54_Cart_Stat  = AS_i_50(6);
    A_54_Cart_Next  = AS_i_50(7);
    A_54_Optic      = AS_i_50(8);
    A_54_Count      = AS_i_50(9);
    A_54_Pist_Bck   = AS_i_50(10);
    A_54_Release_FB = AS_i_50(11);
    A_54_CRoute_In  = AS_i_50(12);
    C_55_Start      = AS_i_50(13);
    C_55_Cart2Del   = AS_i_50(14);
    %Control_50
    C_55_Initialization = Control_50(1);
    C_55_PD_Sort        = Control_50(2);
    C_52_Profibus       = Control_50(3);
    C_55_Start          = Control_50(4);
    C_55_Cart2Del       = Control_50(5);
    %Actuators_50
    F_52_Claw_2_Del  = Actuators_50(1);
    F_52_Claw_2_Cart = Actuators_50(2);
    F_52_Claw_Down   = Actuators_50(3);
    F_52_Close_Claw  = Actuators_50(4);
    F_53_Led_Start   = Actuators_50(5);
    F_53_Led_Reset   = Actuators_50(6);
    F_53_Led_Extra1  = Actuators_50(7);
    F_53_Led_Extra2  = Actuators_50(8);
    F_53_Panel_O4    = Actuators_50(9);
    F_53_Panel_O5    = Actuators_50(10);
    F_53_Panel_O6    = Actuators_50(11);
    F_53_Panel_O7    = Actuators_50(12);
    %Sensors_50
    O_50_Part_Reserve = Sensors_50(1);
    O_50_Claw_Cart    = Sensors_50(2);
    O_50_Claw_Del     = Sensors_50(3);
    O_50_Claw_Reserve = Sensors_50(4);
    O_50_Claw_Low     = Sensors_50(5);
    O_50_Claw_High    = Sensors_50(6);
    O_50_Part_in_Claw = Sensors_50(7);
    O_51_Start        = Sensors_50(8);
    O_51_Stop         = Sensors_50(9);
    O_51_Key_Pos      = Sensors_50(10);
    O_51_Reset        = Sensors_50(11);
    O_51_Panel_I4     = Sensors_50(12);
    O_51_Panel_I5     = Sensors_50(13);
    O_51_Panel_I6     = Sensors_50(14);
    O_51_Panel_I7     = Sensors_50(15);
  state VarDeclaration_20
    entry:
    %Control_20
    C_24_CRoute_In  = Control_20(1);
    C_25_CRoute_In  = Control_20(2);
    C_26_CRoute_In  = Control_20(3);
    C_27_CRoute_In  = Control_20(4);
    C_28_CRoute_In  = Control_20(5);
    C_29_CRoute_In  = Control_20(6);
    C_24_Request    = Control_20(7);
    C_24_CartDel    = Control_20(8);
    C_24_CRoute_Out = Control_20(9);
    C_25_Request    = Control_20(10);
    C_25_CartDel    = Control_20(11);
    C_25_CRoute_Out = Control_20(12);
    C_26_Request    = Control_20(13);
    C_26_CartDel    = Control_20(14);
    C_26_CRoute_Out = Control_20(15);
    C_27_Request    = Control_20(16);
    C_27_CartDel    = Control_20(17);
    C_27_CRoute_Out = Control_20(18);
    C_28_Request    = Control_20(19);
    C_28_CartDel    = Control_20(20);
    C_28_CRoute_Out = Control_20(21);
    C_29_Request    = Control_20(22);
    C_29_CartDel    = Control_20(23);
    C_29_CRoute_Out = Control_20(24);
    %Actuators_20
    F_22_Led_On       = Actuators_20(1);
    F_22_Led_Off      = Actuators_20(2);
    F_22_Conveyor   = Actuators_20(3);
    F_24_Release_FB   = Actuators_20(4);
    F_25_Release_FB   = Actuators_20(5);
    F_26_Release_FB   = Actuators_20(6);
    F_27_Release_FB   = Actuators_20(7);
    F_28_Release_FB   = Actuators_20(8);
    F_29_Release_FB   = Actuators_20(9);
    %Sensors_20
    O_20_On            = Sensors_20(1);
    O_20_Off           = Sensors_20(2);
    O_20_Controler_On  = Sensors_20(3);
    O_24_Cart_Stat     = Sensors_20(4);
    O_24_Cart_Next     = Sensors_20(5);
    O_24_Optic         = Sensors_20(6);
    O_24_Count         = Sensors_20(7);
    O_24_Pist_Bck      = Sensors_20(8);
    O_25_Cart_Stat     = Sensors_20(9);
    O_25_Cart_Next     = Sensors_20(10);
    O_25_Optic         = Sensors_20(11);
    O_25_Count         = Sensors_20(12);
    O_25_Pist_Back     = Sensors_20(13);
    O_26_Cart_Stat     = Sensors_20(14);
    O_26_Cart_Next     = Sensors_20(15);
    O_26_Optic         = Sensors_20(16);
    O_26_Count         = Sensors_20(17);
    O_26_Pist_Back     = Sensors_20(18);
    O_27_Cart_Stat     = Sensors_20(19);
    O_27_Cart_Next     = Sensors_20(20);
    O_27_Optic         = Sensors_20(21);
    O_27_Count         = Sensors_20(22);
    O_27_Pist_Back     = Sensors_20(23);
    O_28_Cart_Stat     = Sensors_20(24);
    O_28_Cart_Next     = Sensors_20(25);
    O_28_Optic         = Sensors_20(26);
    O_28_Count         = Sensors_20(27);
    O_28_Pist_Back     = Sensors_20(28);
    O_29_Cart_Stat     = Sensors_20(29);
    O_29_Cart_Next     = Sensors_20(30);
    O_29_Optic         = Sensors_20(31);
    O_29_Count         = Sensors_20(32);
    O_29_Pist_Back     = Sensors_20(33);
  state VarDeclaration_30
    entry:
    %AS_i_30
    A_34_Request    = AS_i_30(1);
    A_34_No_Cart    = AS_i_30(2);
    A_34_Cart_Full  = AS_i_30(3);
    A_34_CRoute_Out = AS_i_30(4);
    A_32_RoboCartID = AS_i_30(5);
    A_34_Cart_Stat  = AS_i_30(6);
    A_34_Cart_Next  = AS_i_30(7);
    A_34_Optic      = AS_i_30(8);
    A_34_Count      = AS_i_30(9);
    A_34_Pist_Bck   = AS_i_30(10);
    A_34_Release_FB = AS_i_30(11);
    A_34_CRoute_In  = AS_i_30(12);
    %Control_30
    C_30_Robot1   = Control_30(1);
    C_30_Robot2   = Control_30(2);
    C_35_Part_Del = Control_30(3);
    %Actuators_30
    F_33_Led_Start  = Actuators_30(1);
    F_33_Led_Reset  = Actuators_30(2);
    F_33_Led_Extra1 = Actuators_30(3);
    F_33_Led_Extra2 = Actuators_30(4);
    F_33_Spring_Cyl = Actuators_30(5);
    F_33_Cover_Cyl  = Actuators_30(6);
    %Sensors_30
    O_31_Start        = Sensors_30(1);
    O_31_Stop         = Sensors_30(2);
    O_31_Reset        = Sensors_30(3);
    O_31_Part_in_Claw = Sensors_30(4);
    O_31_Orientation  = Sensors_30(5);
    O_32_Sp_Cyl_Bck   = Sensors_30(6);
    O_32_Sp_Cyl_Fwd   = Sensors_30(7);
    O_32_Co_Cyl_Bck   = Sensors_30(8);
    O_32_Co_Cyl_Fwd   = Sensors_30(9);
    O_32_Sp_PickUp    = Sensors_30(10);
    O_32_Co_PickUp    = Sensors_30(11);
    O_32_CoMag_Empty  = Sensors_30(12);
  state Test_Drill
    during:
    C_105_Part_ready
  state ReturnToCart
    during:
    C_95_PD_Cart
  state Start
    during:
    C_24_Request
  state CartToTesting
    during:
    C_24_CartDel
  state GetsPart
    during:
    C_85_Part_Del
  state Identifies Part
    during:
    C_75_Part_Del
    A_74_CRoute_Out
  state CartToHandling2
    during:
    C_25_CartDel
  state DeliverToProcessing
    during:
    C_95_PD_Proc
  state Test_Only
    during:
    C_105_Part_ready
  state CarrinhoParaVision
    during:
    C_26_CartDel
  state Rotation_Only
    during:
    C_105_Part_ready
  (default) -> VarDeclaration_100
  VarDeclaration_90 -> VarDeclaration_80
  VarDeclaration_50 -> VarDeclaration_30
  VarDeclaration_70 -> VarDeclaration_60
  VarDeclaration_30 -> VarDeclaration_20
  VarDeclaration_80 -> VarDeclaration_70
  VarDeclaration_60 -> VarDeclaration_50
  VarDeclaration_100 -> VarDeclaration_90
  Test_Drill -> ReturnToCart : [C_105_Part_ready == true]
  DeliverToProcessing -> Test_Drill [order 1] : [C_95_PD_Proc == true] && [C_105_TestDril == true]
  CartToTesting -> GetsPart : [C_24_CartDel == true]
  Start -> CartToTesting : [C_24_Request == true]
  GetsPart -> Identifies Part : [C_85_Part_Del == true]
  Test_Only -> ReturnToCart : [C_105_Part_ready == true]
  Rotation_Only -> ReturnToCart : [C_105_Part_ready == true]
  DeliverToProcessing -> Test_Only [order 2] : [C_95_PD_Proc == true] && [C_105_Test == true]
  ReturnToCart -> CarrinhoParaVision : [C_95_PD_Cart == true]
  CartToHandling2 -> DeliverToProcessing : [C_25_CartDel == true]
  Identifies Part -> CartToHandling2 : [C_75_Part_Del == true && A_74_CRoute_Out == true ]
  DeliverToProcessing -> Rotation_Only [order 3] : [C_95_PD_Proc == true] && [C_105_Rotation == true]
  data: Control_80 input; Actuators_80 input; Sensors_80 input; AS_i_70 input; Control_70 input; Actuators_70 input; Sensors_70 input; C_82_Profibus local; C_83_RQ_Parts local; C_85_Continuous local; C_85_Counted local; C_85_Initialization local; C_85_Part_Del local; C_85_Single local; C_85_Start local; F_82_Arm_2_Del local; F_82_Arm_2_Mag local; F_82_Pist_Adv local; F_82_Suction_Off local; F_82_Suction_On local; F_83_Led_Extra1 local; F_83_Led_Extra2 local; F_83_Led_Reset local; F_83_Led_Start local; F_83_Panel_O4 local; F_83_Panel_O5 local; F_83_Panel_O6 local; F_83_Panel_O7 local; O_80_Arm_Del local; O_80_Arm_Mag local; O_80_Mag_Empty local; O_80_Mag_Full local; O_80_Part_Stuck local; O_80_Pist_Back local; O_80_Pist_Fwd local; O_81_Key_Pos local; O_81_Panel_I4 local; O_81_Panel_I5 local; O_81_Panel_I6 local; O_81_Panel_I7 local; O_81_Reset local; O_81_Start local; O_81_Stop local; C_75_ID_Delivery1 local; C_75_ID_Delivery2 local; C_75_Identified local; C_75_Identified80 local; C_75_Initialization local; C_75_Part_Del local; C_75_RQ_Delivery1 local; C_75_RQ_Delivery2 local; C_75_RQ_Part_Del local; C_75_RQ_Wrong local; C_75_Requested local; C_75_Requested80 local; F_72_Air_On local; F_72_Eject_Part local; F_72_Elev_Down local; F_72_Elev_Up local; F_73_Led_Extra1 local; F_73_Led_Extra2 local; F_73_Led_Reset local; F_73_Led_Start local; F_73_Panel_O4 local; F_73_Panel_O5 local; F_73_Panel_O6 local; F_73_Panel_O7 local; O_70_Elev_High local; O_70_Elev_Low local; O_70_Pist_Back local; O_70_SInductive local; O_70_SPart local; O_70_SPart_Height local; O_70_SStation local; O_71_Key_Pos local; O_71_Panel_I4 local; O_71_Panel_I5 local; O_71_Panel_I6 local; O_71_Panel_I7 local; O_71_Reset local; O_71_Start local; O_71_Stop local; A_73_TestCartID local; A_74_CRoute_In local; A_74_CRoute_In80 local; A_74_CRoute_Out local; A_74_Cart_Full local; A_74_Cart_Next local; A_74_Cart_Stat local; A_74_Count local; A_74_No_Cart local; A_74_Optic local; A_74_Pist_Bck local; A_74_Release_FB local; A_74_Request local; C_72_Profibus local; AS_i_30 input; AS_i_50 input; AS_i_90 input; Actuators_100 input; Actuators_20 input; Actuators_30 input; Actuators_50 input; Actuators_60 input; Actuators_90 input; Control_100 input; Control_20 input; Control_30 input; Control_50 input; Control_60 input; Control_90 input; Sensors_100 input; Sensors_20 input; Sensors_30 input; Sensors_50 input; Sensors_60 input; Sensors_90 input; A_32_RoboCartID local; A_34_CRoute_In local; A_34_CRoute_Out local; A_34_Cart_Full local; A_34_Cart_Next local; A_34_Cart_Stat local; A_34_Count local; A_34_No_Cart local; A_34_Optic local; A_34_Pist_Bck local; A_34_Release_FB local; A_34_Request local; A_53_SortCartID local; A_54_CRoute_In local; A_54_CRoute_Out local; A_54_Cart_Full local; A_54_Cart_Next local; A_54_Cart_Stat local; A_54_Count local; A_54_No_Cart local; A_54_Optic local; A_54_Pist_Bck local; A_54_Release_FB local; A_54_Request local; A_93_ProcCartID local; A_94_CRoute_In local; A_94_CRoute_Out local; A_94_Cart_Full local; A_94_Cart_Next local; A_94_Cart_Stat local; A_94_Count local; A_94_No_Cart local; A_94_Optic local; A_94_Pist_Bck local; A_94_Release_FB local; A_94_Request local; C_102_Profibus local; C_103_RQ_Turns local; C_105_Initialization local; C_105_Part_ready local; C_105_Rotation local; C_105_Start local; C_105_Test local; C_105_TestDrill local; C_105_Test_Fail local; C_105_Test_Ok local; C_24_CRoute_In local; C_24_CRoute_Out local; C_24_CartDel local; C_24_Request local; C_25_CRoute_In local; C_25_CRoute_Out local; C_25_CartDel local; C_25_Request local; C_26_CRoute_In local; C_26_CRoute_Out local; C_26_CartDel local; C_26_Request local; C_27_CRoute_In local; C_27_CRoute_Out local; C_27_CartDel local; C_27_Request local; C_28_CRoute_In local; C_28_CRoute_Out local; C_28_CartDel local; C_28_Request local; C_29_CRoute_In local; C_29_CRoute_Out local; C_29_CartDel local; C_29_Request local; C_30_Robot1 local; C_30_Robot2 local; C_35_Part_Del local; C_52_Profibus local; C_55_Cart2Del local; C_55_Initialization local; C_55_PD_Sort local; C_55_Start local; C_62_Profibus local; C_65_BRS_Output local; C_65_BSR_Output local; C_65_ID_1 local; C_65_ID_2 local; C_65_Initialization local; C_65_RBS_Output local; C_65_RSB_Output local; C_65_SBR_Output local; C_65_SRB_Output local; C_92_Profibus local; C_95_Cart2Del local; C_95_Del2Cart local; C_95_Initialization local; C_95_PD_Cart local; C_95_PD_Proc local; C_95_Start local; F_102_Drill_Down local; F_102_Drill_On local; F_102_Drill_Pin local; F_102_Drill_Up local; F_102_RT_On local; F_102_Test_Pin local; F_103_Led_Extra1 local; F_103_Led_Extra2 local; F_103_Led_Reset local; F_103_Led_Start local; F_103_Panel_O4 local; F_103_Panel_O5 local; F_103_Panel_O6 local; F_103_Panel_O7 local; F_22_Led_Off local; F_22_Led_On local; F_24_Release_FB local; F_25_Release_FB local; F_26_Release_FB local; F_27_Release_FB local; F_28_Release_FB local; F_29_Release_FB local; F_33_Cover_Cyl local; F_33_Led_Extra1 local; F_33_Led_Extra2 local; F_33_Led_Reset local; F_33_Led_Start local; F_33_Spring_Cyl local; F_52_Claw_2_Cart local; F_52_Claw_2_Del local; F_52_Claw_Down local; F_52_Close_Claw local; F_53_Led_Extra1 local; F_53_Led_Extra2 local; F_53_Led_Reset local; F_53_Led_Start local; F_53_Panel_O4 local; F_53_Panel_O5 local; F_53_Panel_O6 local; F_53_Panel_O7 local; F_62_Conveyor local; F_62_Identify local; F_62_P1 local; F_62_P2 local; F_63_Led_Extra1 local; F_63_Led_Extra2 local; F_63_Led_Reset local; F_63_Led_Start local; F_63_Panel_O4 local; F_63_Panel_O5 local; F_63_Panel_O6 local; F_63_Panel_O7 local; F_92_Claw_2_Cart local; F_92_Claw_2_Del local; F_92_Claw_Down local; F_92_Close_Claw local; F_93_Led_Extra1 local; F_93_Led_Extra2 local; F_93_Led_Reset local; F_93_Led_Start local; F_93_Panel_O4 local; F_93_Panel_O5 local; F_93_Panel_O6 local; F_93_Panel_O7 local; O_100_PDrill_Pos local; O_100_PInit_Pos local; O_100_PTest_Ok local; O_100_PTest_Pos local; O_100_RT_Sensor local; O_100_SDrill_High local; O_100_SDrill_Low local; O_101_Key_Pos local; O_101_Panel_I4 local; O_101_Panel_I5 local; O_101_Panel_I6 local; O_101_Panel_I7 local; O_101_Reset local; O_101_Start local; O_101_Stop local; O_20_Controler_On local; O_20_Off local; O_20_On local; O_24_Cart_Next local; O_24_Cart_Stat local; O_24_Count local; O_24_Optic local; O_24_Pist_Bck local; O_25_Cart_Next local; O_25_Cart_Stat local; O_25_Count local; O_25_Optic local; O_25_Pist_Back local; O_26_Cart_Next local; O_26_Cart_Stat local; O_26_Count local; O_26_Optic local; O_26_Pist_Back local; O_27_Cart_Next local; O_27_Cart_Stat local; O_27_Count local; O_27_Optic local; O_27_Pist_Back local; O_28_Cart_Next local; O_28_Cart_Stat local; O_28_Count local; O_28_Optic local; O_28_Pist_Back local; O_29_Cart_Next local; O_29_Cart_Stat local; O_29_Count local; O_29_Optic local; O_29_Pist_Back local; O_31_Orientation local; O_31_Part_in_Claw local; O_31_Reset local; O_31_Start local; O_31_Stop local; O_32_CoMag_Empty local; O_32_Co_Cyl_Bck local; O_32_Co_Cyl_Fwd local; O_32_Co_PickUp local; O_32_Sp_Cyl_Bck local; O_32_Sp_Cyl_Fwd local; O_32_Sp_PickUp local; O_50_Claw_Cart local; O_50_Claw_Del local; O_50_Claw_High local; O_50_Claw_Low local; O_50_Claw_Reserve local; O_50_Part_Reserve local; O_50_Part_in_Claw local; O_51_Key_Pos local; O_51_Panel_I4 local; O_51_Panel_I5 local; O_51_Panel_I6 local; O_51_Panel_I7 local; O_51_Reset local; O_51_Start local; O_51_Stop local; O_60_Part_Pass local; O_60_SL1_Bck local; O_60_SL1_Fwd local; O_60_SL2_Bck local; O_60_SL2_Fwd local; O_60_SPart local; O_60_SPhoto local; O_60_Slnd local; O_61_Key_Pos local; O_61_Panel_I4 local; O_61_Panel_I5 local; O_61_Panel_I6 local; O_61_Panel_I7 local; O_61_Reset local; O_61_Start local; O_61_Stop local; O_90_Claw_Cart local; O_90_Claw_Del local; O_90_Claw_High local; O_90_Claw_Low local; O_90_Claw_Reserve local; O_90_Part_Reserve local; O_90_Part_in_Claw local; O_91_Key_Pos local; O_91_Panel_I4 local; O_91_Panel_I5 local; O_91_Panel_I6 local; O_91_Panel_I7 local; O_91_Reset local; O_91_Start local; O_91_Stop local; F_22_Conveyor local
